simulink model "DCMotor_M3_ClosedLoopHW"  (R2026b)
settings: Solver=FixedStepDiscrete  StopTime=M3_StopTime  FixedStep=Ts
PreLoadFcn:
  | DCMotorParams;
InitFcn:
  | DCMotorParams;
values from neighbouring files (symbols this model uses):
  Ref_StopTime = Ref_Period*((Ref_Start - Ref_Min)/Ref_Step + 1)    (= 42)    [DCMotorParams.m]
  Ts = 0.01    [DCMotorParams.m]
libraries: simulink x1
settings Model: SILPILModeSetting=veronly  SimulationMode=external  Creator=bence  LastModifiedBy=bence
settings OptimizationCC: DifferentSizesBufferReuse=on  EfficientTunableParamExpr=on  EnhancedBackFolding=on  MaxStackSize=64  OptimizationCustomize=off  OptimizeBlockOrder=speed  PassReuseOutputArgsAs=Individual arguments  RemoveInternalMemoryZeroInit=on  RemoveRootLevelIOMemoryZeroInit=on
settings DebuggingCC: ParameterTunabilityLossMsg=error
settings HardwareCC: ProdHWDeviceType=Atmel->AVR  ProdLargestAtomicFloat=None
settings SFSimCC: MATLABDynamicMemAlloc=off
settings RTWCC: BuildConfiguration=Faster Runs  Description=Embedded Coder  HardwareBoard=Arduino Uno  SystemTargetFile=ert.tlc  TLCOptions=-aInlineSetEventsForThisBaseRateFcn=TLC_FALSE -aSuppressMultiTaskScheduler=TLC_FALSE -aRateBasedStepFcn=1  TemplateMakefile=ert_default_tmf  Toolchain=Arduino AVR
settings CodeAppCC: ForceParamTrailComments=on  IgnoreCustomStorageClasses=off  InsertBlockDesc=on  OperatorAnnotations=on  SFDataObjDesc=on  SimulinkDataObjDesc=on
settings ERTTargetCC: CombineSignalStateStructs=on  ExtMode=on  ExtModeAutomaticAllocSize=off  ExtModeIntrfLevel=Level2 - Open  ExtModeMexFile=ext_xcp  ExtModeStaticAlloc=on  SupportContinuousTime=on  SupportVariableSizeSignals=on

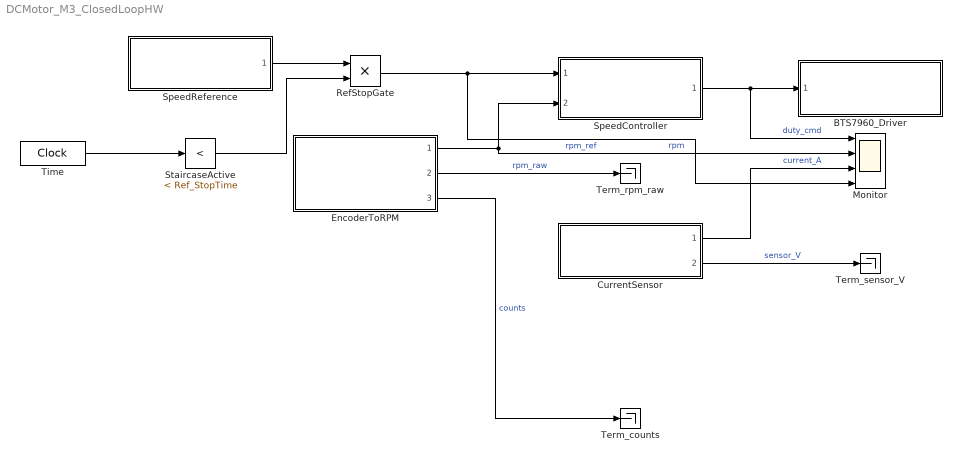
== system DCMotor_M3_ClosedLoopHW ==
  BTS7960_Driver : Subsystem  ReferencedSubsystem=DC7960MDriver
  CurrentSensor : Subsystem  ReferencedSubsystem=CurrentSensor
  EncoderToRPM : Subsystem  ReferencedSubsystem=EncoderToRPM
  Monitor : Scope  NumInputPorts=4
      settings: ActiveDisplayYMinimum=-1883.4976959228516  ActiveDisplayYMaximum=1892.3264312744141
  RefStopGate : Product
  SpeedController : Subsystem  ReferencedSubsystem=SpeedController
  SpeedReference : Subsystem  ReferencedSubsystem=SpeedReference
  StaircaseActive : simulink/Logic and Bit Operations/Compare To Constant  relop=<  const=Ref_StopTime  OutDataTypeStr=boolean
  Term_counts : Terminator
  Term_rpm_raw : Terminator
  Term_sensor_V : Terminator
  Time : DigitalClock  SampleTime=Ts
  wires:
  SpeedController/1 -> BTS7960_Driver/1, Monitor/1  "duty_cmd"
  RefStopGate/1 -> Monitor/4, SpeedController/1  "rpm_ref"
  StaircaseActive/1 -> RefStopGate/2
  Time/1 -> StaircaseActive/1
  SpeedReference/1 -> RefStopGate/1
  EncoderToRPM/1 -> Monitor/2, SpeedController/2  "rpm"
  EncoderToRPM/2 -> Term_rpm_raw/1  "rpm_raw"
  EncoderToRPM/3 -> Term_counts/1  "counts"
  CurrentSensor/1 -> Monitor/3  "current_A"
  CurrentSensor/2 -> Term_sensor_V/1  "sensor_V"
